simulink model "sim_realimentacion_por_VE"  (R2021a)
settings: Solver=VariableStepAuto  StartTime=0.0  StopTime=5  RelTol=1e-3
values from neighbouring files (symbols this model uses):
  A_d = I + A*Ts    [realimentacion_estados.m]
  B_d = B*Ts    [realimentacion_estados.m]
  C_d = C    [realimentacion_estados.m]
  F = 1/(C*inv(eye(2)-(A_d+B_d*K))*B_d)    [realimentacion_estados.m]
  K = -place(A_d,B_d,polos)    [realimentacion_estados.m]
  Ts = 0.02    [realimentacion_estados.m]
settings Model: Creator=mdiaz  LastModifiedBy=mdiaz

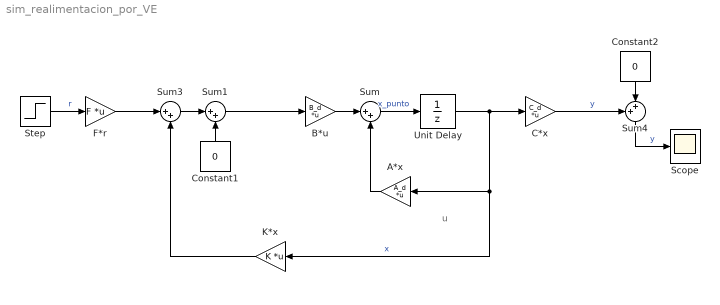
== system sim_realimentacion_por_VE ==
  note: u
  A*x : Gain  Gain=A_d  Multiplication=Matrix(K*u)
  B*u : Gain  Gain=B_d  Multiplication=Matrix(K*u)
  C*x : Gain  Gain=C_d  Multiplication=Matrix(K*u)
  Constant1 : Constant  Value=0
  Constant2 : Constant  Value=0
  F*r : Gain  Gain=F  Multiplication=Matrix(K*u)
  K*x : Gain  Gain=K  Multiplication=Matrix(K*u)
  Scope : Scope
  Step : Step  After=10  SampleTime=Ts
  Sum : Sum  Inputs=|++
  Sum1 : Sum  Inputs=|++
  Sum3 : Sum  Inputs=|++
  Sum4 : Sum  Inputs=++|
  Unit Delay : UnitDelay  SampleTime=Ts  HasFrameUpgradeWarning=on
  wires:
  B*u/1 -> Sum/1
  A*x/1 -> Sum/2
  Sum/1 -> Unit Delay/1  "x_punto"
  Unit Delay/1 -> C*x/1, K*x/1, A*x/1  "x"
  Sum3/1 -> Sum1/1
  Sum1/1 -> B*u/1
  Constant1/1 -> Sum1/2
  C*x/1 -> Sum4/1  "y"
  K*x/1 -> Sum3/2
  F*r/1 -> Sum3/1
  Step/1 -> F*r/1  "r"
  Sum4/1 -> Scope/1  "y"
  Constant2/1 -> Sum4/2
